simulink library "Controller_Lib"  (R2025a)
settings: Solver=VariableStepAuto  StartTime=0.0  StopTime=10.0  RelTol=1e-3  EnableMultiTasking=on
undefined symbols (not defined in the file or in its folder): Scissor_Lift_Param
libraries: fl_lib x32, nesl_utility x2, slpidlib x1, fl_ps_legacy_lib x1
Description:
  | Copyright 2016-2025 The MathWorks, Inc.
settings Model: Creator=smiller  LastModifiedBy=smiller
settings SolverCC: AlgebraicLoopSolver=TrustRegion
settings DataIOCC: LimitDataPoints=on  ReturnWorkspaceOutputs=off
settings OptimizationCC: ReuseModelBlockBuffer=off  LifeSpan=inf
settings DebuggingCC: UnconnectedInputMsg=warning  UnconnectedOutputMsg=warning  UnconnectedLineMsg=warning  AllowSymbolicDim=off  PregeneratedLibrarySubsystemCodeDiagnostic=none  SFUnexpectedBacktrackingDiag=warning  SFNoUnconditionalDefaultTransitionDiag=warning  SFExecutionAtInitializationDiag=none  ArithmeticOperatorsInVariantConditions=warning
settings HardwareCC: ProdWordSize=32.0
settings ModelReferenceCC: EnableRefExpFcnMdlSchedulingChecks=on  PropagateSignalLabelsOutOfModel=off
settings SFSimCC: SimUseLocalCustomCode=off  CustomCodeUndefinedFunction=UseInterfaceOnly
settings RTWCC: RTWUseLocalCustomCode=off  GPUComputeCapability=3.5  DLArmComputeVersion=19.05
settings CodeAppCC: StateflowObjectComments=on
settings GRTTargetCC: TargetLangStandard=C89/C90 (ANSI)
settings ConfigComp: CovMetricSettings=dw  CovSaveCumulativeToWorkspaceVar=on  CovSaveSingleToWorkspaceVar=on  CovExternalEMLEnable=off

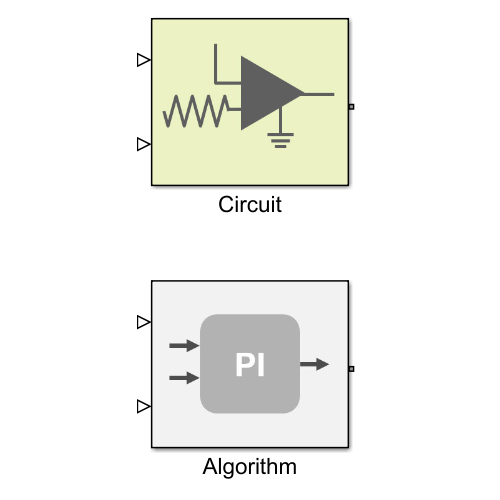
[thumbnail: Simulink's stored preview of the top-level diagram]
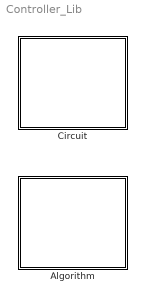
== system Controller_Lib ==
  Algorithm : Subsystem  VariantControl=Algorithm
      mask Display: image('Algorithm_Controller_IMAGE.jpg')
  Circuit : Subsystem  VariantControl=Circuit
      mask Display: image('Analog_PI_Controller_IMAGE.jpg')

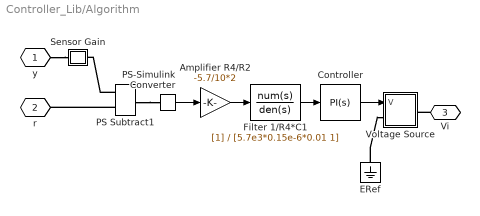
== system Controller_Lib/Algorithm ==
  Amplifier R4/R2 : Gain  Gain=-5.7/10*2
  Controller : slpidlib/PID Controller  Controller=PI  Form=Parallel  TimeDomain=Continuous-time  UseExternalTs=off  SampleTime=-1  IntegratorMethod=Forward Euler  FilterMethod=Forward Euler  ControllerParametersSource=internal  P=20/10  I=1/(10e3*100e-6)/10  UseKiTs=off  D=0  UseExternalDerivativeSource=off  N=100  UseFilter=on  TunerSelectOption=Transfer Function Based (PID Tuner App)  InitialConditionSource=internal  InitialConditionForIntegrator=0  InitialConditionForFilter=0  DifferentiatorICPrevScaledInput=0  ExternalReset=none  TrackingMode=off  Kt=1  LimitOutput=off  SatLimitsSource=internal  UpperSaturationLimit=inf  LowerSaturationLimit=-inf  LinearizeAsGain=on  AntiWindupMode=none  Kb=1  LimitIntegrator=off  UpperIntegratorSaturationLimit=inf  LowerIntegratorSaturationLimit=-inf  POutMin=[]  POutMax=[]  IOutMin=[]  IOutMax=[]  DOutMin=[]  DOutMax=[]  NOutMin=[]  NOutMax=[]  SumOutMin=[]  SumOutMax=[]  SaturationOutMin=[]  SaturationOutMax=[]  PParamMin=[]  PParamMax=[]  IParamMin=[]  IParamMax=[]  DParamMin=[]  DParamMax=[]  NParamMin=[]  NParamMax=[]  KbParamMin=[]  KbParamMax=[]  KtParamMin=[]  KtParamMax=[]  KbOutMin=[]  KbOutMax=[]  KtOutMin=[]  KtOutMax=[]  IntegratorOutMin=[]  IntegratorOutMax=[]  FilterOutMin=[]  FilterOutMax=[]  SumI1OutMin=[]  SumI1OutMax=[]  SumI2OutMin=[]  SumI2OutMax=[]  SumI3OutMin=[]  SumI3OutMax=[]  SumI4OutMin=[]  SumI4OutMax=[]  SumDOutMin=[]  SumDOutMax=[]  DifferentiatorOutMin=[]  DifferentiatorOutMax=[]  FilterDiffOutCoefMin=[]  FilterDiffOutCoefMax=[]  ReciprocalOutMin=[]  ReciprocalOutMax=[]  SumDenOutMin=[]  SumDenOutMax=[]  SumNumOutMin=[]  SumNumOutMax=[]  DivideOutMin=[]  DivideOutMax=[]  UdiffTsProdOutMin=[]  UdiffTsProdOutMax=[]  NTsProdOutMin=[]  NTsProdOutMax=[]  UintegralTsProdOutMin=[]  UintegralTsProdOutMax=[]  UngainTsProdOutMin=[]  UngainTsProdOutMax=[]  ClampingZeroOutDataTypeStr=Inherit: Inherit via back propagation  ClampingZeroOutMin=[]  ClampingZeroOutMax=[]  FilterDenConstantOutDataTypeStr=Inherit: Inherit via back propagation  FilterDenConstantOutMin=[]  FilterDenConstantOutMax=[]  PCopyOutDataTypeStr=Inherit: Inherit via back propagation  PCopyOutMin=[]  PCopyOutMax=[]  NCopyOutDataTypeStr=Inherit: Inherit via back propagation  NCopyOutMin=[]  NCopyOutMax=[]  IntegratorContinuousStateAttributes=''  IntegratorStateMustResolveToSignalObject=off  IntegratorRTWStateStorageClass=Auto  FilterContinuousStateAttributes=''  FilterStateMustResolveToSignalObject=off  FilterRTWStateStorageClass=Auto  ParallelPVariant=InternalParameters  IdealPVariant=Disabled  IVariant=InternalParameters  DVariant=Disabled  IntegratorVariant=Continuous  SatVariant=Disabled  AWVariant=Passthrough  PCopyVariant=Disabled  TRVariant=Disabled  FdbkBlocksVariant=Forward  IdealPFdbkVariant=Disabled  SatFdbkVariant=Disabled  DerivativeFilterVariant=Disabled  NVariant=Disabled  NCopyVariant=Disabled_SignalSpec  FilterICVariant=Disabled  IntegratorICVariant=InternalICs  ExternalResetVariant=Disabled  TRSumVariant=Passthrough  SumFdbkVariant=Disabled  SumVariant=Sum_PI  TsampFilterVariant=InternalTs  TsampNgainVariant=Passthrough  TsampIntegralVariant=Disabled_SignalSpec  ExternalSaturationOutDataTypeStr=Inherit: Same as second input  DerivativeSourceVariant=Disabled  PreIntVariant=InternalPreInt
  ERef : fl_lib/Electrical/Electrical Elements/Electrical Reference
  Filter 1/R4*C1 : TransferFcn  Denominator=[5.7e3*0.15e-6*0.01 1]
  PS Subtract1 : fl_lib/Physical Signals/Functions/PS Subtract
  PS-Simulink Converter : nesl_utility/PS-Simulink Converter  PhysicalDomain=network_engine_domain  SubClassName=ps_output  LeftPortType=input  RightPortType=output  PseudoPeriodic=off  Frequencies=[]  VectorFormat=1-D array  Unit=V  AffineConversion=off
  Sensor Gain : Subsystem
      mask Display: disp('G')
  Voltage Source : Subsystem
  y : PMIOPort  Tag=PMCPort  Side=Left
  r : PMIOPort  Tag=PMCPort  Port=2  Side=Left
  Vi : PMIOPort  Port=3  Side=Right
  wires:
  PS-Simulink Converter/1 -> Amplifier R4/R2/1
  Amplifier R4/R2/1 -> Filter 1/R4*C1/1
  Filter 1/R4*C1/1 -> Controller/1
  Controller/1 -> Voltage Source/1(V)
  connections:
  PS Subtract1/RConn1 -- PS-Simulink Converter/LConn1
  ERef/LConn1 -- Voltage Source/LConn1
  PS Subtract1/LConn2 -- r/RConn1
  y/RConn1 -- Sensor Gain/LConn1
  Vi/RConn1 -- Voltage Source/RConn1
  PS Subtract1/LConn1 -- Sensor Gain/RConn1

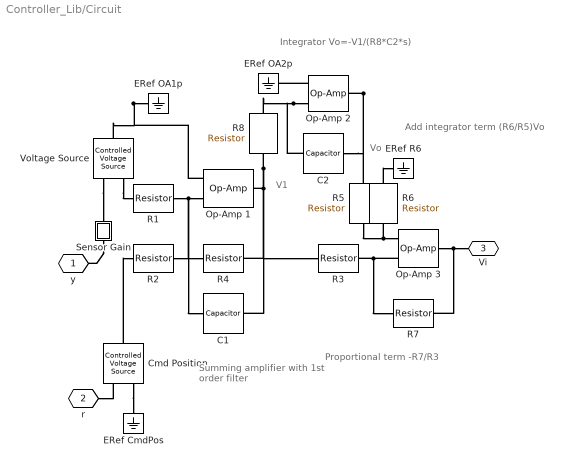
== system Controller_Lib/Circuit ==
  note: V1
  note: Vo
  note: Add integrator
      | term (R6/R5)Vo
  note: Proportional
      | term -R7/R3
  note: Integrator
      | Vo=-V1/(R8*C2*s)
  note: Summing amplifier
      | with 1st order filter
  C1 : fl_lib/Electrical/Electrical Elements/Capacitor  c=0.15e-06 F  r=1e-06 Ohm  g=0 1/Ohm  i_specify=off  i_priority=High  i=0 A  i_nominal_specify=off  i_nominal_value=1  i_nominal_unit=A  v_specify=off  v_priority=High  v=0 V  v_nominal_specify=off  v_nominal_value=1  v_nominal_unit=V  vc_specify=on  vc_priority=High  vc=0 V  vc_nominal_specify=off  vc_nominal_value=1  vc_nominal_unit=V
  C2 : fl_lib/Electrical/Electrical Elements/Capacitor  c=100e-06*100 F  r=1e-06 Ohm  g=0 1/Ohm  i_specify=off  i_priority=High  i=0 A  i_nominal_specify=off  i_nominal_value=1  i_nominal_unit=A  v_specify=off  v_priority=High  v=0 V  v_nominal_specify=off  v_nominal_value=1  v_nominal_unit=V  vc_specify=on  vc_priority=High  vc=0 V  vc_nominal_specify=off  vc_nominal_value=1  vc_nominal_unit=V
  Cmd Position : fl_lib/Electrical/Electrical Sources/Controlled Voltage Source
  ERef CmdPos : fl_lib/Electrical/Electrical Elements/Electrical Reference
  ERef OA1p : fl_lib/Electrical/Electrical Elements/Electrical Reference
  ERef OA2p : fl_lib/Electrical/Electrical Elements/Electrical Reference
  ERef R6 : fl_lib/Electrical/Electrical Elements/Electrical Reference
  Op-Amp 1 : fl_lib/Electrical/Electrical Elements/Op-Amp  outI_specify=off  outI_priority=High  outI=0 A  outI_nominal_specify=off  outI_nominal_value=1  outI_nominal_unit=A
  Op-Amp 2 : fl_lib/Electrical/Electrical Elements/Op-Amp  outI_specify=off  outI_priority=High  outI=0 A  outI_nominal_specify=off  outI_nominal_value=1  outI_nominal_unit=A
  Op-Amp 3 : fl_lib/Electrical/Electrical Elements/Op-Amp  outI_specify=off  outI_priority=High  outI=0 A  outI_nominal_specify=off  outI_nominal_value=1  outI_nominal_unit=A
  R{1..3,5..6,8} (6 alike) : fl_lib/Electrical/Electrical Elements/Resistor  R=10e3 Ohm  i_specify=off  i_priority=High  i=0 A  i_nominal_specify=off  i_nominal_value=1  i_nominal_unit=A  v_specify=off  v_priority=High  v=0 V  v_nominal_specify=off  v_nominal_value=1  v_nominal_unit=V
  R4 : fl_lib/Electrical/Electrical Elements/Resistor  R=5.7e3*2 Ohm  i_specify=off  i_priority=High  i=0 A  i_nominal_specify=off  i_nominal_value=1  i_nominal_unit=A  v_specify=off  v_priority=High  v=0 V  v_nominal_specify=off  v_nominal_value=1  v_nominal_unit=V
  R7 : fl_lib/Electrical/Electrical Elements/Resistor  R=20e3 Ohm  i_specify=off  i_priority=High  i=0 A  i_nominal_specify=off  i_nominal_value=1  i_nominal_unit=A  v_specify=off  v_priority=High  v=0 V  v_nominal_specify=off  v_nominal_value=1  v_nominal_unit=V
  Sensor Gain : Subsystem
      mask Display: disp('G')
  Voltage Source : fl_lib/Electrical/Electrical Sources/Controlled Voltage Source
  y : PMIOPort  Tag=PMCPort  Side=Left
  r : PMIOPort  Tag=PMCPort  Port=2  Side=Left
  Vi : PMIOPort  Port=3  Side=Right
  connections:
  Sensor Gain/LConn1 -- y/RConn1
  Voltage Source/RConn1 -- Sensor Gain/RConn1
  Op-Amp 2/LConn1 -- ERef OA2p/LConn1
  R6/RConn1 -- ERef R6/LConn1
  Cmd Position/RConn2 -- ERef CmdPos/LConn1
  Cmd Position/LConn1 -- R2/LConn1
  Voltage Source/RConn2 -- R1/LConn1
  R3/RConn1 -- R7/LConn1 -- Op-Amp 3/LConn2
  Op-Amp 3/LConn1 -- R6/LConn1 -- R5/RConn1
  ERef OA1p/LConn1 -- Voltage Source/LConn1 -- Op-Amp 1/LConn1
  Op-Amp 2/RConn1 -- R5/LConn1 -- C2/RConn1
  Op-Amp 2/LConn2 -- C2/LConn1 -- R8/RConn1
  R8/LConn1 -- Op-Amp 1/RConn1 -- R3/LConn1 -- C1/RConn1 -- R4/RConn1
  Op-Amp 1/LConn2 -- C1/LConn1 -- R4/LConn1 -- R2/RConn1 -- R1/RConn1
  Op-Amp 3/RConn1 -- R7/RConn1 -- Vi/RConn1
  r/RConn1 -- Cmd Position/RConn1

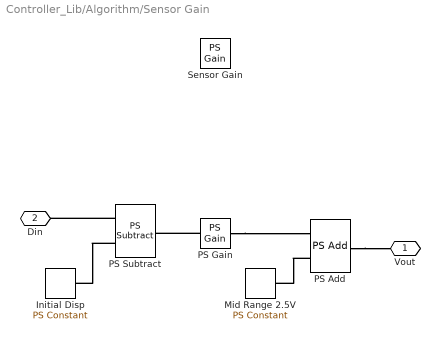
== system Controller_Lib/Algorithm/Sensor Gain ==
  Initial Disp : fl_lib/Physical Signals/Sources/PS Constant  constant=Scissor_Lift_Param.Initial_Cyl_Ext mm
  Mid Range 2.5V : fl_lib/Physical Signals/Sources/PS Constant  constant=2.5 V
  PS Add : fl_lib/Physical Signals/Functions/PS Add
  PS Gain : fl_lib/Physical Signals/Functions/PS Gain  gain=Scissor_Lift_Param.Sensor_Gain V/m
  PS Subtract : fl_lib/Physical Signals/Functions/PS Subtract
  Sensor Gain : fl_ps_legacy_lib/Legacy Physical Signals/Functions/PS Gain  gain=Scissor_Lift_Param.Sensor_Gain
  Vout : PMIOPort  Side=Right
  Din : PMIOPort  Port=2  Side=Left
  connections:
  PS Subtract/LConn1 -- Din/RConn1
  PS Gain/LConn1 -- PS Subtract/RConn1
  PS Add/RConn1 -- Vout/RConn1
  PS Subtract/LConn2 -- Initial Disp/RConn1
  PS Gain/RConn1 -- PS Add/LConn1
  PS Add/LConn2 -- Mid Range 2.5V/RConn1

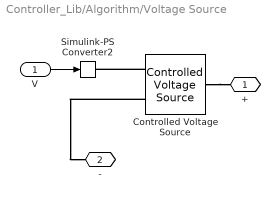
== system Controller_Lib/Algorithm/Voltage Source ==
  V : Inport
  Controlled Voltage Source : fl_lib/Electrical/Electrical Sources/Controlled Voltage Source
  Simulink-PS Converter2 : nesl_utility/Simulink-PS Converter  PhysicalDomain=network_engine_domain  SubClassName=ps_input  LeftPortType=input  RightPortType=output  PseudoPeriodic=off  Frequencies=[]  NoiseDistribution=none  NoiseParameters=[]  Unit=V  AffineConversion=off  FilteringAndDerivatives=filter  SimscapeFilterOrder=1  InputFilterTimeConstant=0.005  UdotUserProvided=1
  + : PMIOPort  Side=Right
  - : PMIOPort  Port=2  Side=Left
  wires:
  V/1 -> Simulink-PS Converter2/1
  connections:
  Controlled Voltage Source/RConn1 -- Simulink-PS Converter2/RConn1
  Controlled Voltage Source/LConn1 -- +/RConn1
  Controlled Voltage Source/RConn2 -- -/RConn1

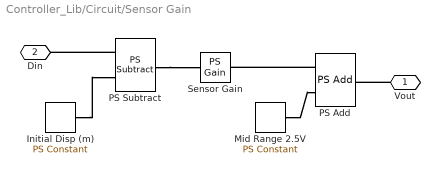
== system Controller_Lib/Circuit/Sensor Gain ==
  Initial Disp (m) : fl_lib/Physical Signals/Sources/PS Constant  constant=Scissor_Lift_Param.Initial_Cyl_Ext*1e-3 m
  Mid Range 2.5V : fl_lib/Physical Signals/Sources/PS Constant  constant=2.5 V
  PS Add : fl_lib/Physical Signals/Functions/PS Add
  PS Subtract : fl_lib/Physical Signals/Functions/PS Subtract
  Sensor Gain : fl_lib/Physical Signals/Functions/PS Gain  gain=Scissor_Lift_Param.Sensor_Gain V/m
  Vout : PMIOPort  Side=Right
  Din : PMIOPort  Port=2  Side=Left
  connections:
  Mid Range 2.5V/RConn1 -- PS Add/LConn2
  PS Add/LConn1 -- Sensor Gain/RConn1
  Initial Disp (m)/RConn1 -- PS Subtract/LConn2
  Vout/RConn1 -- PS Add/RConn1
  PS Subtract/RConn1 -- Sensor Gain/LConn1
  PS Subtract/LConn1 -- Din/RConn1
